simulink model "dgira"  (R2025b)
settings: Solver=FixedStepAuto  StartTime=0.0  StopTime=10.0  FixedStep=0.001  RelTol=1e-3
PreLoadFcn:
  | m = 10;
  | k = 100;
  | r = 0.05;
InitFcn:
  | m = 10;
  | k = 100;
  | r = 0.05;
libraries: fl_lib x7, nesl_utility x3
settings Model: Creator=GUIA  LastModifiedBy=GUIA

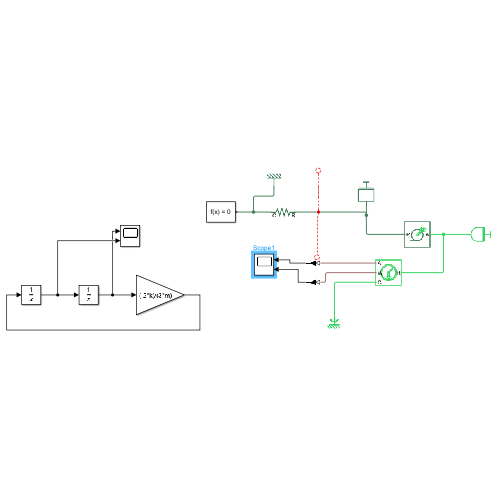
[thumbnail: Simulink's stored preview of the top-level diagram]
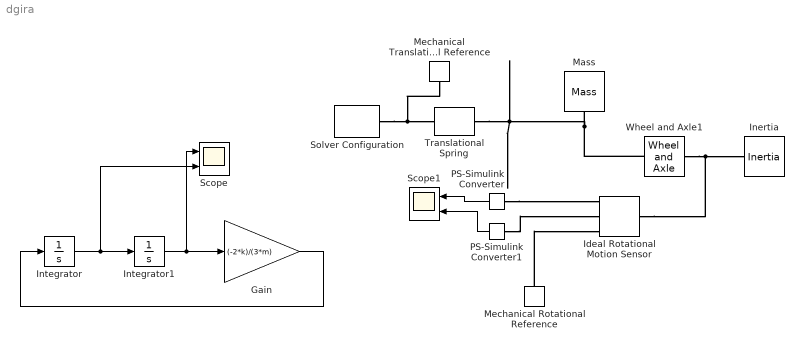
== system dgira ==
  Gain : Gain  Gain=(-2*k)/(3*m)
  Ideal Rotational Motion Sensor : fl_lib/Mechanical/Mechanical Sensors/Ideal Rotational Motion Sensor  reference=foundation.enum.MeasurementReference.difference  acceleration_port=false  velocity_port=true  position_port=true  wrap_angle=false  offset=0 rad
  Inertia : fl_lib/Mechanical/Rotational Elements/Inertia  inertia=0.5 * 10 * 0.05*0.05 kg*m^2  num_ports=foundation.enum.numPorts2.one  w_specify=on  w_priority=High  w=2 rad/s  w_nominal_specify=off  w_nominal_value=1  w_nominal_unit=rad/s  t_specify=off  t_priority=None  t=0 N*m  t_nominal_specify=off  t_nominal_value=1  t_nominal_unit=N*m
  Integrator : Integrator  InitialCondition=2
  Integrator1 : Integrator
  Mass : fl_lib/Mechanical/Translational Elements/Mass  mass=10 kg  num_ports=foundation.enum.numPorts2.one  v_specify=off  v_priority=High  v=0 m/s  v_nominal_specify=off  v_nominal_value=1  v_nominal_unit=m/s  f_specify=off  f_priority=None  f=0 N  f_nominal_specify=off  f_nominal_value=1  f_nominal_unit=N
  Mechanical Rotational Reference : fl_lib/Mechanical/Rotational Elements/Mechanical Rotational Reference
  Mechanical Translational Reference : fl_lib/Mechanical/Translational Elements/Mechanical Translational Reference
  PS-Simulink Converter : nesl_utility/PS-Simulink Converter  PhysicalDomain=network_engine_domain  SubClassName=ps_output  LeftPortType=input  RightPortType=output  PseudoPeriodic=off  Frequencies=[]  VectorFormat=inherit  Unit=inherit  AffineConversion=off
  PS-Simulink Converter1 : nesl_utility/PS-Simulink Converter  PhysicalDomain=network_engine_domain  SubClassName=ps_output  LeftPortType=input  RightPortType=output  PseudoPeriodic=off  Frequencies=[]  VectorFormat=inherit  Unit=inherit  AffineConversion=off
  Scope : Scope  NumInputPorts=2
      settings: ActiveDisplayYMinimum=-2.4999998273801629  ActiveDisplayYMaximum=2.499999980820018
  Scope1 : Scope  NumInputPorts=2
      settings: ActiveDisplayYMinimum=-1.052716325737231  ActiveDisplayYMaximum=1.4998467992627698
  Solver Configuration : nesl_utility/Solver Configuration  PhysicalDomain=network_engine_domain  SubClassName=solver  LeftPortType=input  RightPortType=generic  Tones=[]  Harmonics=[]  SimulateNoise=off  Profile=off  UseLocalSampling=off  EnableSwitchedLinearOptims=on  FrequencyDomain=off  UseCCode=off  RelTol=0.001  AbsTol=0.001  MinStep=1e-09  ToWorkspace=off  RevertToSquareIcSolve=off  NumHomotopyIterations=100  PhasorMode=off  PhasorModeNumHarmonics=1  ConsistencySolver=NEWTON_XTOL_AFTER_FTOL  IndexReductionMethod=DerivativeReplacement  DoDC=off  ResidualTolerance=1e-09  ConsistencyTolSource=GLOBAL  ConsistencyAbsTol=0.001  ConsistencyRelTol=0.001  ConsistencyTolFactor=0.001  UseLocalSolver=off  LocalSolverChoice=NE_BACKWARD_EULER_ADVANCER  ResolveIndetEquations=on  FunctionEvalNumThread=1  LocalSolverSampleTime=0.001  DoFixedCost=off  MaxNonlinIter=3  MaxModeIter=2  ComputeImpulses=off  ImpulseIterations=2  LinearAlgebra=auto  LinearAlgebraNumThread=0  EquationFormulation=NE_TIME_EF  DelaysMemoryBudget=1024  AutomaticFiltering=on  FilteringTimeConstant=0.001  PartitionStorageMethod=AS_NEEDED  PartitionMemoryBudget=1024  PartitionMethod=ROBUST  MultibodyUseLocalSolver=off  MultibodyLocalSolverChoice=ODE1  MultibodyLocalSolverSampleTime=0.001
  Translational Spring : fl_lib/Mechanical/Translational Elements/Translational Spring  spr_rate=100 N/m  v_specify=off  v_priority=None  v=0 m/s  v_nominal_specify=off  v_nominal_value=1  v_nominal_unit=m/s  f_specify=off  f_priority=None  f=0 N  f_nominal_specify=off  f_nominal_value=1  f_nominal_unit=N  x_specify=off  x_priority=High  x=0 m  x_nominal_specify=off  x_nominal_value=1  x_nominal_unit=m
  Wheel and Axle1 : fl_lib/Mechanical/Mechanisms/Wheel and Axle  R=0.05 m  or=foundation.enum.DriveOrientation.Positive  t_specify=off  t_priority=None  t=0 N*m  t_nominal_specify=off  t_nominal_value=1  t_nominal_unit=N*m  f_specify=off  f_priority=None  f=0 N  f_nominal_specify=off  f_nominal_value=1  f_nominal_unit=N
  wires:
  Integrator/1 -> Scope/2, Integrator1/1
  Integrator1/1 -> Scope/1, Gain/1
  Gain/1 -> Integrator/1
  PS-Simulink Converter/1 -> Scope1/1
  PS-Simulink Converter1/1 -> Scope1/2
  connections:
  Wheel and Axle1/RConn1 -- Mass/LConn1 -- Translational Spring/LConn1
  Wheel and Axle1/LConn1 -- Inertia/LConn1 -- Ideal Rotational Motion Sensor/LConn1
  Mechanical Rotational Reference/LConn1 -- Ideal Rotational Motion Sensor/RConn1
  PS-Simulink Converter/LConn1 -- Ideal Rotational Motion Sensor/RConn3
  PS-Simulink Converter1/LConn1 -- Ideal Rotational Motion Sensor/RConn2
  Solver Configuration/RConn1 -- Mechanical Translational Reference/LConn1 -- Translational Spring/RConn1
